simulink model "jacobian_path_planning"  (R2024a)
settings: Solver=ode45  StartTime=0.0  StopTime=simulation_time  RelTol=1e-3
InitFcn:
  | initial_q = evalin('base', 'initial_q');
values from neighbouring files (symbols this model uses):
  a0 = evalin('base', 'a0')    [setup_project.m]
  a1 = evalin('base', 'a1')    [setup_project.m]
  a2 = evalin('base', 'a2')    [setup_project.m]
  a3 = evalin('base', 'a3')    [setup_project.m]
  L1 = evalin('base', 'L1')    [setup_project.m]
  L2 = evalin('base', 'L2')    [setup_project.m]
  target = evalin('base', 'target')    [run_example.m]
undefined symbols (not defined in the file or in its folder): algorithm_selection, Kp, max_joint_speed, model_selection
settings Model: Creator=asialalala  LastModifiedBy=asialalala

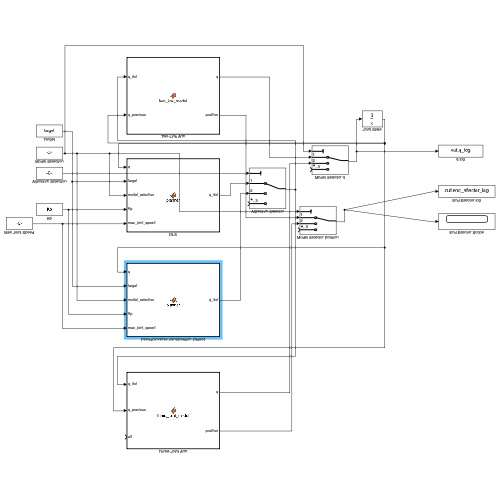
[thumbnail: Simulink's stored preview of the top-level diagram]
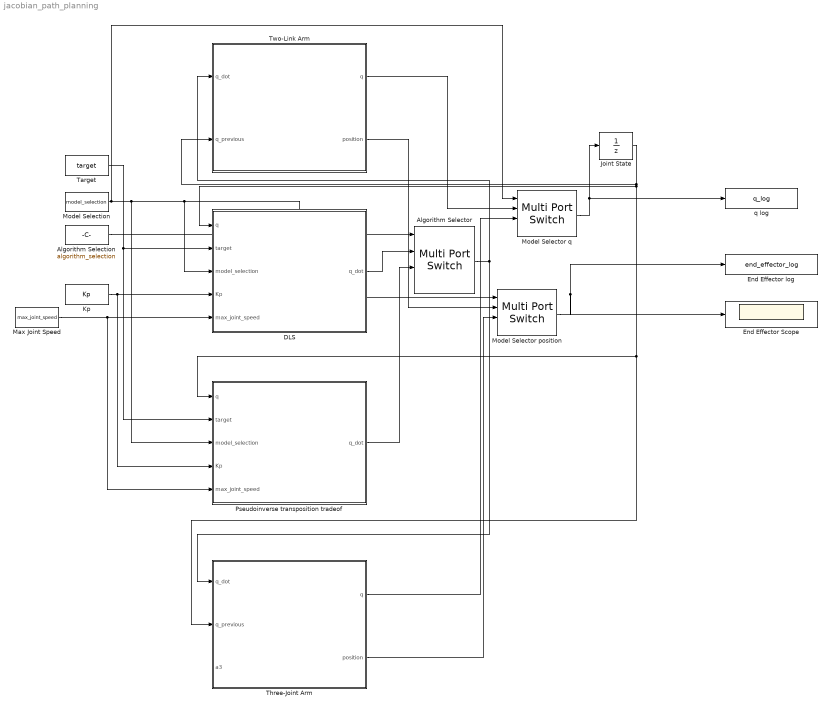
== system jacobian_path_planning ==
  Algorithm Selection : Constant  Value=algorithm_selection
  Algorithm Selector : MultiPortSwitch  SaturateOnIntegerOverflow=off  InputSameDT=off
  DLS : MATLAB Function  TreatAsAtomicUnit=on
  End Effector Scope : Scope
  End Effector log : ToWorkspace  VariableName=end_effector_log  SaveFormat=Structure With Time  SampleTime=-1
  Joint State : UnitDelay  InitialCondition=initial_q  SampleTime=0.01  HasFrameUpgradeWarning=on
  Kp : Constant  Value=Kp
  Max Joint Speed : Constant  Value=max_joint_speed
  Model Selection : Constant  Value=model_selection
  Model Selector position : MultiPortSwitch  SaturateOnIntegerOverflow=off  InputSameDT=off
  Model Selector q : MultiPortSwitch  SaturateOnIntegerOverflow=off  InputSameDT=off
  Pseudoinverse transposition tradeof : MATLAB Function  TreatAsAtomicUnit=on
  Target : Constant  Value=target
  Three-Joint Arm : MATLAB Function  TreatAsAtomicUnit=on
  Two-Link Arm : MATLAB Function  TreatAsAtomicUnit=on
  q log : ToWorkspace  VariableName=q_log  SaveFormat=Structure With Time  SampleTime=-1
  wires:
  Algorithm Selection/1 -> Algorithm Selector/1
  DLS/1(q_dot) -> Algorithm Selector/2
  Pseudoinverse transposition tradeof/1(q_dot) -> Algorithm Selector/3
  Algorithm Selector/1 -> Three-Joint Arm/1(q_dot), Two-Link Arm/1(q_dot)
  Joint State/1 -> DLS/1(q), Pseudoinverse transposition tradeof/1(q), Three-Joint Arm/2(q_previous), Two-Link Arm/2(q_previous)
  Model Selection/1 -> Model Selector position/1, DLS/3(model_selection), Pseudoinverse transposition tradeof/3(model_selection), Model Selector q/1
  Two-Link Arm/1(q) -> Model Selector q/2
  Three-Joint Arm/1(q) -> Model Selector q/3
  Two-Link Arm/2(position) -> Model Selector position/2
  Three-Joint Arm/2(position) -> Model Selector position/3
  Model Selector q/1 -> Joint State/1, q log/1
  Target/1 -> Pseudoinverse transposition tradeof/2(target), DLS/2(target)
  Kp/1 -> Pseudoinverse transposition tradeof/4(Kp), DLS/4(Kp)
  Max Joint Speed/1 -> Pseudoinverse transposition tradeof/5(max_joint_speed), DLS/5(max_joint_speed)
  Model Selector position/1 -> End Effector log/1, End Effector Scope/1

== matlab function jacobian_path_planning/Pseudoinverse transposition tradeof ==
  data: q input; q_dot output; target input; model_selection input; Kp input; max_joint_speed input; L1 parameter; L2 parameter; a0 parameter; a1 parameter; a2 parameter; a3 parameter
function q_dot = planner(q, target, model_selection, Kp, max_joint_speed, L1, L2, a0, a1, a2, a3)
%#codegen
position = zeros(3,1); J = zeros(3,3);
if model_selection == 1
    q12 = q(1:2);
    position(1:2) = two_link_position(q12, L1, L2);
    J(1:2,1:2) = two_link_jacobian(q12, L1, L2);
else
    position = three_joint_position(q, a0, a1, a2, a3);
    J = three_joint_jacobian(q, a0, a1, a2, a3);
end
error = target - position;
command = Kp * error;

A = J*J'
%% lambda calculation
    % 1. funckja wymierna
    ad = abs(det(A))
    lambda = ad/(1+ad);
    % 2. tw. Hadamana SŁABE BO CZASEM DZIELI PRZEZ 0
    % ad = abs(det(A));
    % m = prod(vecnorm(A,2,2));
    % if ad ~= 0
    %    lambda = ad/m;
    % else
    %     lambda = 0;
    % end
    % 3. condition number
    % ae = eig(A);
    % lambda = abs(min(ae)/max(ae));

%%
I = eye(size(J,1));
q_dot_task = J' * ((A*lambda + (1-lambda)*I) \ command);
q_dot = q_dot_task;
% q_dot = min(max(q_dot, -max_joint_speed), max_joint_speed); limit jon spee
end

function position = two_link_position(q, L1, L2)
position = [L1*cos(q(1))+L2*cos(q(1)+q(2)); L1*sin(q(1))+L2*sin(q(1)+q(2))];
end

function J = two_link_jacobian(q, L1, L2)
J = [-L1*sin(q(1))-L2*sin(q(1)+q(2)), -L2*sin(q(1)+q(2)); ...
     L1*cos(q(1))+L2*cos(q(1)+q(2)), L2*cos(q(1)+q(2))];
end

function position = three_joint_position(q, a0, a1, a2, a3)
A = a1+a2*cos(q(2))+a3*cos(q(2)+q(3));
position = [cos(q(1))*A; sin(q(1))*A; a0+a2*sin(q(2))+a3*sin(q(2)+q(3))];
end

function J = three_joint_jacobian(q, a0, a1, a2, a3)
h = 1e-6; J = zeros(3,3);
for k = 1:3
    qp=q; qm=q; qp(k)=qp(k)+h; qm(k)=qm(k)-h;
    J(:,k)=(three_joint_position(qp,a0,a1,a2,a3)-three_joint_position(qm,a0,a1,a2,a3))/(2*h);
end
end

== matlab function jacobian_path_planning/DLS ==
  data: q input; q_dot output; target input; model_selection input; Kp input; max_joint_speed input; L1 parameter; L2 parameter; a0 parameter; a1 parameter; a2 parameter; a3 parameter
function q_dot = planner(q, target, model_selection, Kp, max_joint_speed, L1, L2, a0, a1, a2, a3)
%#codegen
position = zeros(3,1); J = zeros(3,3);
if model_selection == 1
    q12 = q(1:2);
    position(1:2) = two_link_position(q12, L1, L2);
    J(1:2,1:2) = two_link_jacobian(q12, L1, L2);
else
    position = three_joint_position(q, a0, a1, a2, a3);
    J = three_joint_jacobian(q, a0, a1, a2, a3);
end
error = target - position;
command = Kp * error;
lambda = 0.05;
q_dot_task = J' * ((J*J' + lambda^2*eye(size(J,1))) \ command);
q_dot = q_dot_task;
% q_dot = min(max(q_dot, -max_joint_speed), max_joint_speed); limit joint
% speed
end

function position = two_link_position(q, L1, L2)
position = [L1*cos(q(1))+L2*cos(q(1)+q(2)); L1*sin(q(1))+L2*sin(q(1)+q(2))];
end

function J = two_link_jacobian(q, L1, L2)
J = [-L1*sin(q(1))-L2*sin(q(1)+q(2)), -L2*sin(q(1)+q(2)); ...
     L1*cos(q(1))+L2*cos(q(1)+q(2)), L2*cos(q(1)+q(2))];
end

function position = three_joint_position(q, a0, a1, a2, a3)
A = a1+a2*cos(q(2))+a3*cos(q(2)+q(3));
position = [cos(q(1))*A; sin(q(1))*A; a0+a2*sin(q(2))+a3*sin(q(2)+q(3))];
end

function J = three_joint_jacobian(q, a0, a1, a2, a3)
h = 1e-6; J = zeros(3,3);
for k = 1:3
    qp=q; qm=q; qp(k)=qp(k)+h; qm(k)=qm(k)-h;
    J(:,k)=(three_joint_position(qp,a0,a1,a2,a3)-three_joint_position(qm,a0,a1,a2,a3))/(2*h);
end
end

== matlab function jacobian_path_planning/Two-Link Arm ==
  data: q_dot input; q output; q_previous input; position output; L1 parameter; L2 parameter; a0 parameter; a1 parameter; a2 parameter; a3 parameter
function [q, position] = two_link_model(q_dot, q_previous, L1, L2, a0, a1, a2, a3)
%#codegen
q=q_previous+0.01*q_dot; q(3)=0;
position=[L1*cos(q(1))+L2*cos(q(1)+q(2)); L1*sin(q(1))+L2*sin(q(1)+q(2)); 0];
end

== matlab function jacobian_path_planning/Three-Joint Arm ==
  data: q_dot input; q output; q_previous input; position output; a3 input; L1 parameter; L2 parameter; a0 parameter; a1 parameter; a2 parameter
function [q, position] = three_joint_model(q_dot, q_previous, a3, L1, L2, a0, a1, a2)
%#codegen
q=q_previous+0.01*q_dot;
A=a1+a2*cos(q(2))+a3*cos(q(2)+q(3));
position=[cos(q(1))*A; sin(q(1))*A; a0+a2*sin(q(2))+a3*sin(q(2)+q(3))];
end
